simulink model "app_speed"  (R2023a)
settings: Solver=FixedStepDiscrete  StartTime=0.0  StopTime=8  RelTol=1e-3  EnableMultiTasking=on
undefined symbols (not defined in the file): ctrl_limits, PU_System, Ts_speed
libraries: focLib x8, simulink x5, svdschedulerlib x4, c2838xlib x1
Description:
  | Anwendung Drehzahlregelung (CarPediem). Komponenten aus focLib.
settings Model: ExtModeTrigDuration=8  Creator=baris  LastModifiedBy=Student
settings SolverCC: AutoInsertRateTranBlk=on
settings DataIOCC: LimitDataPoints=on  SaveFormat=Array  SaveOutput=off  SaveTime=off  ReturnWorkspaceOutputs=off
settings OptimizationCC: DefaultUnderspecifiedDataType=single  EnhancedBackFolding=on  PassReuseOutputArgsAs=Individual arguments  MaxStackSize=1024  OptimizeBlockOrder=speed  DifferentSizesBufferReuse=on  DenormalBehavior=FlushToZero  EfficientTunableParamExpr=on
settings DebuggingCC: ReadBeforeWriteMsg=DisableAll  WriteAfterWriteMsg=DisableAll  WriteAfterReadMsg=DisableAll  SignalResolutionControl=TryResolveAllWithWarning  InheritedTsInSrcMsg=none  MultiTaskDSMMsg=none  MultiTaskCondExecSysMsg=none  TasksWithSamePriorityMsg=none  SigSpecEnsureSampleTimeMsg=none  IntegerOverflowMsg=none  ParameterPrecisionLossMsg=none  FcnCallInpInsideContextMsg=warning  UnconnectedInputMsg=warning  UnconnectedOutputMsg=warning  UnconnectedLineMsg=warning  IntegerSaturationMsg=none
settings HardwareCC: ProdBitPerChar=16  ProdBitPerInt=16  ProdBitPerPointer=32  ProdBitPerSizeT=32  ProdBitPerPtrDiffT=32  ProdLargestAtomicInteger=Integer  ProdLargestAtomicFloat=None  ProdWordSize=16  ProdLongLongMode=on  ProdHWDeviceType=Texas Instruments->C2000  HardwareBoardFeatureSet=SoCBlockset
settings ModelReferenceCC: EnableRefExpFcnMdlSchedulingChecks=on  PropagateSignalLabelsOutOfModel=off
settings SFSimCC: MATLABDynamicMemAlloc=off
settings RTWCC: Description=Embedded Coder  SystemTargetFile=ert.tlc  HardwareBoard=TI F2838x  TemplateMakefile=ert_default_tmf  CustomDefine=-DCARPEDIEM_PIN_CORRECTION  Toolchain=Texas Instruments Code Composer Studio - EABI (C2000)
settings RTWCC: CustomInclude=|
  | ../../protocol/include
  | ../../protocol/include/focp
  | ../../firmware
settings RTWCC: CustomSource=|
  | ../../protocol/src/focp.c
  | ../../protocol/src/focp_dev.c
  | ../../firmware/focp_target.c
  | ../../firmware/focp_c28x.c
settings CodeAppCC: ForceParamTrailComments=on  IgnoreCustomStorageClasses=off  OperatorAnnotations=on  SimulinkDataObjDesc=on  SFDataObjDesc=on  InsertBlockDesc=on
settings ERTTargetCC: CodeReplacementLibrary=TI C28x  ExtModeTransport=4  ExtModeStaticAlloc=on  ExtModeAutomaticAllocSize=off  ExtModeStaticAllocSize=10000  ExtModeMexFile=ext_xcp  ExtModeIntrfLevel=Level2 - Open
settings ConfigComp: CovEnable=on  RecordCoverage=on  CovModelRefEnable=on

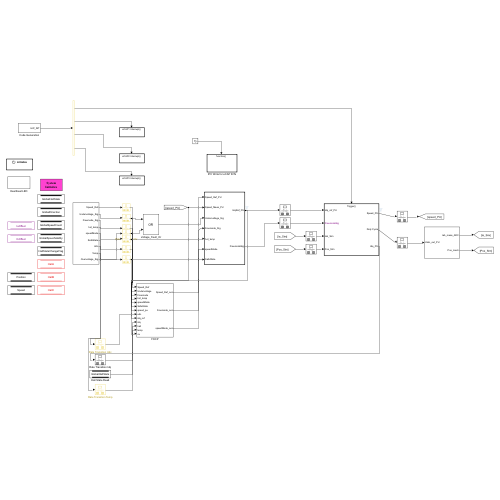
[thumbnail: Simulink's stored preview of the top-level diagram]
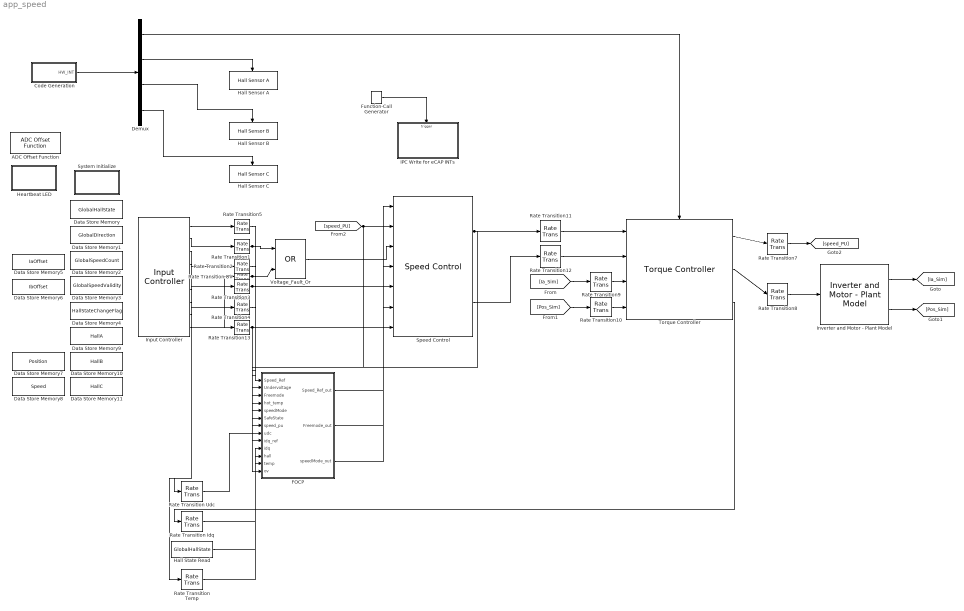
== system app_speed ==
  ADC Offset Function : focLib/ADC Offset Function  SystemSampleTime=-1  VariantActivationTime=update diagram  Latency=0  AutoFrameSizeCalculation=off
  Code Generation : Subsystem
  Data Store Memory : DataStoreMemory  DataStoreName=GlobalHallState  WriteAfterWriteMsg=warning  ShowAdditionalParam=off
  Data Store Memory1 : DataStoreMemory  DataStoreName=GlobalDirection  WriteAfterWriteMsg=warning  ShowAdditionalParam=off
  Data Store Memory10 : DataStoreMemory  DataStoreName=HallB  WriteAfterWriteMsg=warning  ShowAdditionalParam=off
  Data Store Memory11 : DataStoreMemory  DataStoreName=HallC  WriteAfterWriteMsg=warning  ShowAdditionalParam=off
  Data Store Memory2 : DataStoreMemory  DataStoreName=GlobalSpeedCount  WriteAfterWriteMsg=warning  ShowAdditionalParam=off
  Data Store Memory3 : DataStoreMemory  DataStoreName=GlobalSpeedValidity  WriteAfterWriteMsg=warning  ShowAdditionalParam=off
  Data Store Memory4 : DataStoreMemory  DataStoreName=HallStateChangeFlag  WriteAfterWriteMsg=warning  ShowAdditionalParam=off
  Data Store Memory5 : DataStoreMemory  DataStoreName=IaOffset  WriteAfterWriteMsg=warning  ShowAdditionalParam=off
  Data Store Memory6 : DataStoreMemory  DataStoreName=IbOffset  WriteAfterWriteMsg=warning  ShowAdditionalParam=off
  Data Store Memory7 : DataStoreMemory  DataStoreName=Position  WriteAfterWriteMsg=warning  ShowAdditionalParam=off
  Data Store Memory8 : DataStoreMemory  DataStoreName=Speed  WriteAfterWriteMsg=warning  ShowAdditionalParam=off
  Data Store Memory9 : DataStoreMemory  DataStoreName=HallA  WriteAfterWriteMsg=warning  ShowAdditionalParam=off
  Demux : Demux
  FOCP : Subsystem
  Function-Call Generator : simulink/Ports & Subsystems/Function-Call Generator  sample_time=-1  numberOfIterations=1  DisallowWideOutput=off
  Hall Sensor A : focLib/Hall Sensor A  SystemSampleTime=-1  VariantActivationTime=update diagram  Latency=0  AutoFrameSizeCalculation=off
  Hall Sensor B : focLib/Hall Sensor B  SystemSampleTime=-1  VariantActivationTime=update diagram  Latency=0  AutoFrameSizeCalculation=off
  Hall Sensor C : focLib/Hall Sensor C  SystemSampleTime=-1  VariantActivationTime=update diagram  Latency=0  AutoFrameSizeCalculation=off
  Hall State Read : DataStoreRead  DataStoreName=GlobalHallState  SampleTime=Ts_speed  IndexOptions=Index vector (dialog)  Indices=1  OutputSizes=1
  Heartbeat LED : Subsystem
  IPC Write for eCAP INTs : Subsystem
  Input Controller : focLib/Input Controller  SystemSampleTime=-1  VariantActivationTime=update diagram  Latency=0  AutoFrameSizeCalculation=off
  Inverter and Motor - Plant Model : focLib/Inverter and Motor - Plant Model  SystemSampleTime=-1  VariantActivationTime=update diagram  Latency=0  AutoFrameSizeCalculation=off
  Rate Transition Idq : RateTransition  Deterministic=off  OutPortSampleTime=Ts_speed
  Rate Transition OV : RateTransition  Deterministic=off  OutPortSampleTime=Ts_speed
  Rate Transition Temp : RateTransition  Deterministic=off  OutPortSampleTime=Ts_speed
  Rate Transition Udc : RateTransition  Deterministic=off  OutPortSampleTime=Ts_speed
  Rate Transition1 : RateTransition  Deterministic=off  OutPortSampleTime=Ts_speed
  Rate Transition{9..12} (4 alike) : RateTransition  Deterministic=off
  Rate Transition{2..4,13} (4 alike) : RateTransition  Integrity=off  Deterministic=off  OutPortSampleTime=Ts_speed
  Rate Transition5 : RateTransition  Deterministic=off  OutPortSampleTime=Ts_speed
  Rate Transition7 : RateTransition  Deterministic=off  OutPortSampleTime=Ts_speed
  Rate Transition8 : RateTransition  Deterministic=off  OutPortSampleTime=Ts_simulink
  Speed Control : focLib/Speed Control  SystemSampleTime=Ts_speed  VariantActivationTime=update diagram  Latency=0  AutoFrameSizeCalculation=off
  System Initialize : Subsystem  mask(System Initialize){ShowInLibBrowser=0}
      mask prompts: ShowInLibBrowser "Simulink:masks:CustCodeMaskParam1_MP"
      settings: CopyFcn=cccopyfcn(gcb)  OpenFcn=ccopenfcn('System Initialize Function')
      mask Help: eval('feval(''rtwprivate'',''rtwhelpview'',''rtw_sys_initialize_block'')');
      mask DialogControl ShowInLibBrowser Prompt: Mask Parameter 1:
      mask Display: disp('System\nInitialize');
  Torque Controller : focLib/Torque Controller  SystemSampleTime=-1  VariantActivationTime=update diagram  Latency=0  AutoFrameSizeCalculation=off
  Voltage_Fault_Or : Logic  Operator=OR  AllPortsSameDT=off  OutDataTypeStr=boolean
  wires:
  Code Generation/1(HW_INT) -> Demux/1
  Demux/1 -> Torque Controller/Trigger
  Torque Controller/1 -> Rate Transition7/1
  [speed_PU] -> Speed Control/2, FOCP/7(speed_pu)
  Input Controller/1 -> Rate Transition5/1
  Input Controller/2 -> Rate Transition1/1
  Input Controller/3 -> Rate Transition2/1
  Input Controller/4 -> Rate Transition3/1
  Input Controller/5 -> Rate Transition4/1
  Rate Transition1/1 -> FOCP/2(Undervoltage), Voltage_Fault_Or/1
  Rate Transition3/1 -> Speed Control/5, FOCP/4(hot_temp)
  Rate Transition4/1 -> FOCP/5(speedMode)
  Inverter and Motor - Plant Model/1 -> [Ia_Sim]
  Inverter and Motor - Plant Model/2 -> [Pos_Sim]
  Torque Controller/2 -> Rate Transition8/1
  Rate Transition8/1 -> Inverter and Motor - Plant Model/1
  Rate Transition10/1 -> Torque Controller/4
  [Pos_Sim] -> Rate Transition10/1
  [Ia_Sim] -> Rate Transition9/1
  Rate Transition9/1 -> Torque Controller/3
  Speed Control/1 -> Rate Transition11/1, FOCP/9(idq_ref)
  Speed Control/2 -> Rate Transition12/1
  Rate Transition11/1 -> Torque Controller/1
  Rate Transition12/1 -> Torque Controller/2
  Rate Transition7/1 -> [speed_PU]
  Input Controller/6 -> Rate Transition13/1
  Rate Transition13/1 -> Speed Control/7, FOCP/6(SafeState)
  Demux/2 -> Hall Sensor A/Trigger
  Demux/3 -> Hall Sensor B/Trigger
  Demux/4 -> Hall Sensor C/Trigger
  Function-Call Generator/1 -> IPC Write for eCAP INTs/Trigger
  Rate Transition5/1 -> FOCP/1(Speed_Ref)
  Rate Transition2/1 -> FOCP/3(Freemode)
  FOCP/1(Speed_Ref_out) -> Speed Control/1
  FOCP/2(Freemode_out) -> Speed Control/4
  Input Controller/7 -> Rate Transition Udc/1
  Torque Controller/3 -> Rate Transition Idq/1
  Rate Transition Udc/1 -> FOCP/8(udc)
  Rate Transition Idq/1 -> FOCP/10(idq)
  Hall State Read/1 -> FOCP/11(hall)
  Input Controller/8 -> Rate Transition Temp/1
  Rate Transition Temp/1 -> FOCP/12(temp)
  Input Controller/9 -> Rate Transition OV/1
  Rate Transition OV/1 -> Voltage_Fault_Or/2, FOCP/13(ov)
  Voltage_Fault_Or/1 -> Speed Control/3
  FOCP/3(speedMode_out) -> Speed Control/6

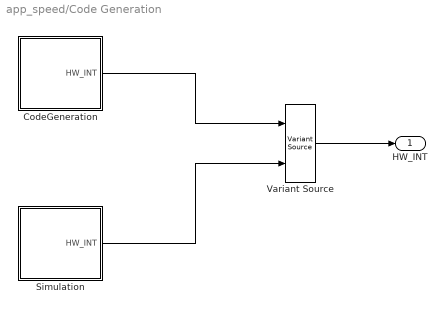
== system app_speed/Code Generation ==
  CodeGeneration : Subsystem
  Simulation : Subsystem
  Variant Source : VariantSource  VariantControlMode=sim codegen switching  OutputFunctionCall=on
  HW_INT : Outport
  wires:
  Variant Source/1 -> HW_INT/1
  CodeGeneration/1(HW_INT) -> Variant Source/1
  Simulation/1(HW_INT) -> Variant Source/2

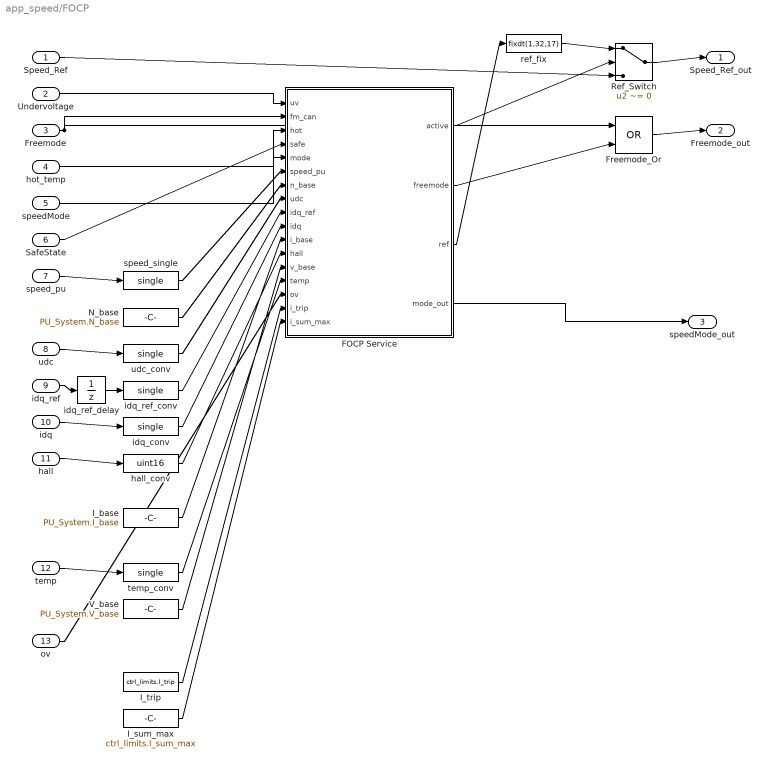
== system app_speed/FOCP ==
  Speed_Ref : Inport
  Undervoltage : Inport  Port=2
  Freemode : Inport  Port=3
  hot_temp : Inport  Port=4
  speedMode : Inport  Port=5
  SafeState : Inport  Port=6
  speed_pu : Inport  Port=7
  udc : Inport  Port=8
  idq_ref : Inport  Port=9
  idq : Inport  Port=10
  hall : Inport  Port=11
  temp : Inport  Port=12
  ov : Inport  Port=13
  FOCP Service : MATLAB Function  TreatAsAtomicUnit=on
  Freemode_Or : Logic  Operator=OR  AllPortsSameDT=off  OutDataTypeStr=boolean
  I_base : Constant  Value=PU_System.I_base  OutDataTypeStr=single  SampleTime=-1
  I_sum_max : Constant  Value=ctrl_limits.I_sum_max  OutDataTypeStr=single  SampleTime=-1
  I_trip : Constant  Value=ctrl_limits.I_trip  OutDataTypeStr=single  SampleTime=-1
  N_base : Constant  Value=PU_System.N_base  OutDataTypeStr=single  SampleTime=-1
  Ref_Switch : Switch  Criteria=u2 ~= 0  SaturateOnIntegerOverflow=off  InputSameDT=off
  V_base : Constant  Value=PU_System.V_base  OutDataTypeStr=single  SampleTime=-1
  hall_conv : DataTypeConversion  OutDataTypeStr=uint16  SaturateOnIntegerOverflow=off  RndMeth=Floor
  idq_conv : DataTypeConversion  OutDataTypeStr=single  SaturateOnIntegerOverflow=off  RndMeth=Floor
  idq_ref_conv : DataTypeConversion  OutDataTypeStr=single  SaturateOnIntegerOverflow=off  RndMeth=Floor
  idq_ref_delay : UnitDelay  SampleTime=-1  HasFrameUpgradeWarning=on
  ref_fix : DataTypeConversion  OutDataTypeStr=fixdt(1,32,17)  RndMeth=Nearest  SaturateOnIntegerOverflow=off
  speed_single : DataTypeConversion  OutDataTypeStr=single  SaturateOnIntegerOverflow=off  RndMeth=Floor
  temp_conv : DataTypeConversion  OutDataTypeStr=single  SaturateOnIntegerOverflow=off  RndMeth=Floor
  udc_conv : DataTypeConversion  OutDataTypeStr=single  SaturateOnIntegerOverflow=off  RndMeth=Floor
  Speed_Ref_out : Outport
  Freemode_out : Outport  Port=2
  speedMode_out : Outport  Port=3
  wires:
  Undervoltage/1 -> FOCP Service/1(uv)
  Freemode/1 -> FOCP Service/2(fm_can), Freemode_Or/1
  hot_temp/1 -> FOCP Service/3(hot)
  SafeState/1 -> FOCP Service/4(safe)
  speedMode/1 -> FOCP Service/5(mode)
  speed_pu/1 -> speed_single/1
  speed_single/1 -> FOCP Service/6(speed_pu)
  N_base/1 -> FOCP Service/7(n_base)
  FOCP Service/3(ref) -> ref_fix/1
  ref_fix/1 -> Ref_Switch/1
  FOCP Service/1(active) -> Ref_Switch/2
  Speed_Ref/1 -> Ref_Switch/3
  Ref_Switch/1 -> Speed_Ref_out/1
  FOCP Service/2(freemode) -> Freemode_Or/2
  Freemode_Or/1 -> Freemode_out/1
  udc/1 -> udc_conv/1
  udc_conv/1 -> FOCP Service/8(udc)
  idq_ref_conv/1 -> FOCP Service/9(idq_ref)
  idq/1 -> idq_conv/1
  idq_conv/1 -> FOCP Service/10(idq)
  I_base/1 -> FOCP Service/11(i_base)
  hall/1 -> hall_conv/1
  hall_conv/1 -> FOCP Service/12(hall)
  idq_ref/1 -> idq_ref_delay/1
  idq_ref_delay/1 -> idq_ref_conv/1
  temp/1 -> temp_conv/1
  V_base/1 -> FOCP Service/13(v_base)
  temp_conv/1 -> FOCP Service/14(temp)
  ov/1 -> FOCP Service/15(ov)
  I_trip/1 -> FOCP Service/16(i_trip)
  I_sum_max/1 -> FOCP Service/17(i_sum_max)
  FOCP Service/4(mode_out) -> speedMode_out/1

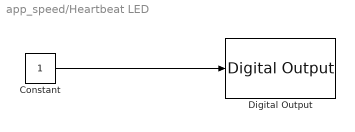
== system app_speed/Heartbeat LED ==
  Constant : Constant  SampleTime=0.5
  Digital Output : c2838xlib/Digital Output  GPIO_Number=GPIO56~GPIO63  GPIO_Bit0=on  GPIO_BIT0_Toggle=on  GPIO_Bit1=off  GPIO_BIT1_Toggle=off  GPIO_Bit2=off  GPIO_BIT2_Toggle=off  GPIO_Bit3=off  GPIO_BIT3_Toggle=off  GPIO_Bit4=off  GPIO_BIT4_Toggle=off  GPIO_Bit5=off  GPIO_BIT5_Toggle=off  GPIO_Bit6=off  GPIO_BIT6_Toggle=off  GPIO_Bit7=off  GPIO_BIT7_Toggle=off
  wires:
  Constant/1 -> Digital Output/1

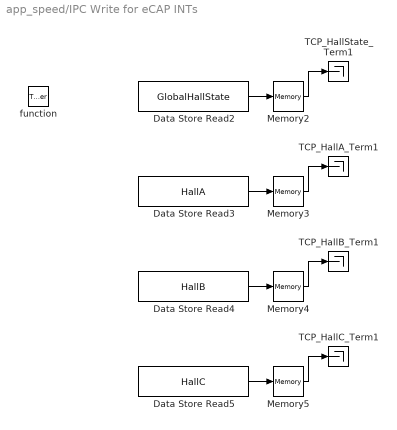
== system app_speed/IPC Write for eCAP INTs ==
  function : TriggerPort  TriggerType=function-call  VariantControl=(inherit)
  Data Store Read2 : DataStoreRead  DataStoreName=GlobalHallState  IndexOptions=Index vector (dialog)  Indices=1  OutputSizes=1
  Data Store Read3 : DataStoreRead  DataStoreName=HallA  IndexOptions=Index vector (dialog)  Indices=1  OutputSizes=1
  Data Store Read4 : DataStoreRead  DataStoreName=HallB  IndexOptions=Index vector (dialog)  Indices=1  OutputSizes=1
  Data Store Read5 : DataStoreRead  DataStoreName=HallC  IndexOptions=Index vector (dialog)  Indices=1  OutputSizes=1
  Memory{2..5} (4 alike) : Memory  InheritSampleTime=on
  TCP_HallA_Term1 : Terminator
  TCP_HallB_Term1 : Terminator
  TCP_HallC_Term1 : Terminator
  TCP_HallState_Term1 : Terminator
  wires:
  Data Store Read2/1 -> Memory2/1
  Data Store Read3/1 -> Memory3/1
  Data Store Read4/1 -> Memory4/1
  Data Store Read5/1 -> Memory5/1
  Memory3/1 -> TCP_HallA_Term1/1
  Memory4/1 -> TCP_HallB_Term1/1
  Memory5/1 -> TCP_HallC_Term1/1
  Memory2/1 -> TCP_HallState_Term1/1

== system app_speed/System Initialize ==

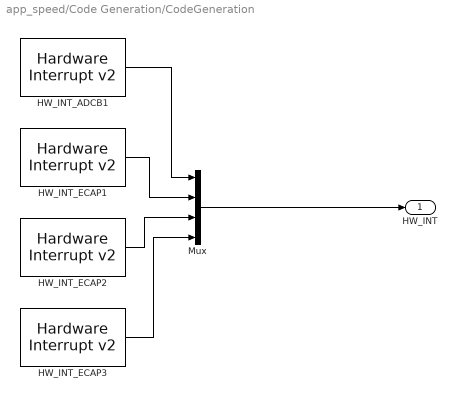
== system app_speed/Code Generation/CodeGeneration ==
  HW_INT_ADCB1 : svdschedulerlib/Hardware Interrupt v2  ISRGroup=ADC - Analog to Digital Converter  ISRName=ADCA1_INT  ISRNumber=32  NumEventsToServe=1  EventsList={'on','EOC event','1';'off','Overflow event','2';'off','Custom event','3'}  SelectedEvents={'event1'}  TaskPriority=30  DisablePreemption=off  ClearInterruptFlagsAtEndOfEvent=on  InterruptDefinitionFile=$(TARGET_ROOT)/registry/interrupts/F2837xS_interrupts.xml  HardwareBoard=F2837x  EnableSimPort=off
      settings: LibrarySourceBlock=c2000lib/Scheduling/Hardware Interrupt
  HW_INT_ECAP1 : svdschedulerlib/Hardware Interrupt v2  ISRGroup=ADC - Analog to Digital Converter  ISRName=ADCA1_INT  ISRNumber=32  NumEventsToServe=1  EventsList={'on','EOC event','1';'off','Overflow event','2';'off','Custom event','3'}  SelectedEvents={'event1'}  TaskPriority=25  DisablePreemption=on  ClearInterruptFlagsAtEndOfEvent=on  InterruptDefinitionFile=$(TARGET_ROOT)/registry/interrupts/F2837xS_interrupts.xml  HardwareBoard=F2837x  EnableSimPort=off
      settings: LibrarySourceBlock=c2000lib/Scheduling/Hardware Interrupt
  HW_INT_ECAP2 : svdschedulerlib/Hardware Interrupt v2  ISRGroup=ADC - Analog to Digital Converter  ISRName=ADCA1_INT  ISRNumber=32  NumEventsToServe=1  EventsList={'on','EOC event','1';'off','Overflow event','2';'off','Custom event','3'}  SelectedEvents={'event1'}  TaskPriority=25  DisablePreemption=on  ClearInterruptFlagsAtEndOfEvent=on  InterruptDefinitionFile=$(TARGET_ROOT)/registry/interrupts/F2837xS_interrupts.xml  HardwareBoard=F2837x  EnableSimPort=off
      settings: LibrarySourceBlock=c2000lib/Scheduling/Hardware Interrupt
  HW_INT_ECAP3 : svdschedulerlib/Hardware Interrupt v2  ISRGroup=ADC - Analog to Digital Converter  ISRName=ADCA1_INT  ISRNumber=32  NumEventsToServe=1  EventsList={'on','EOC event','1';'off','Overflow event','2';'off','Custom event','3'}  SelectedEvents={'event1'}  TaskPriority=25  DisablePreemption=on  ClearInterruptFlagsAtEndOfEvent=on  InterruptDefinitionFile=$(TARGET_ROOT)/registry/interrupts/F2837xS_interrupts.xml  HardwareBoard=F2837x  EnableSimPort=off
      settings: LibrarySourceBlock=c2000lib/Scheduling/Hardware Interrupt
  Mux : Mux
  HW_INT : Outport
  wires:
  HW_INT_ECAP2/1 -> Mux/3
  HW_INT_ECAP1/1 -> Mux/2
  HW_INT_ECAP3/1 -> Mux/4
  HW_INT_ADCB1/1 -> Mux/1
  Mux/1 -> HW_INT/1

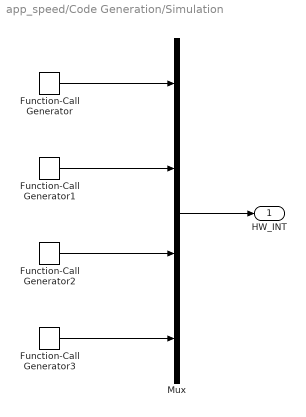
== system app_speed/Code Generation/Simulation ==
  Function-Call Generator{,1..3} (4 alike) : simulink/Ports & Subsystems/Function-Call Generator  sample_time=T_pwm  numberOfIterations=1  DisallowWideOutput=off
  Mux : Mux
  HW_INT : Outport
  wires:
  Mux/1 -> HW_INT/1
  Function-Call Generator/1 -> Mux/1
  Function-Call Generator1/1 -> Mux/2
  Function-Call Generator2/1 -> Mux/3
  Function-Call Generator3/1 -> Mux/4

== matlab function app_speed/FOCP/FOCP Service ==
  data: uv input; active output boolean; fm_can input; hot input; safe input; mode input; speed_pu input; n_base input; freemode output boolean; ref output single; udc input; idq_ref input size=2; idq input size=2; i_base input; hall input; v_base input; temp input; ov input; i_trip input; i_sum_max input; mode_out output
function [active, freemode, ref, mode_out] = focp_service(uv, fm_can, hot, safe, mode, speed_pu, n_base, udc, idq_ref, idq, i_base, hall, v_base, temp, ov, i_trip, i_sum_max)
% FOCP fuer FOC Studio, nur im erzeugten Code (firmware/focp_c28x.c). Simulation: inaktiv,
% speedMode wird unveraendert durchgereicht.
% idq wird nicht mehr benutzt (Stroeme kommen aus focp_c28x_isr im Stromregler-Interrupt).
active = false; freemode = false; ref = single(0); mode_out = mode;
if coder.target('Rtw')
    coder.cinclude('focp_c28x.h');
    a = uint16(0); f = uint16(0); r = single(0); md = uint16(0);
    iref = single(idq_ref);
    coder.ceval('focp_c28x_step', uint16(uv), uint16(ov), uint16(fm_can), uint16(hot), uint16(safe), ...
        uint16(mode), single(speed_pu), single(n_base), single(udc), coder.rref(iref), ...
        single(i_base), single(v_base), single(temp), uint16(hall), single(i_trip), ...
        single(i_sum_max), coder.wref(a), coder.wref(f), coder.wref(r), coder.wref(md));
    active = a ~= 0; freemode = f ~= 0; ref = r; mode_out = cast(md, 'like', mode);
end
end
